simulink model "blok_net_dIt"  (R2024b)
settings: Solver=VariableStepAuto  StartTime=0.0  StopTime=10.0  RelTol=1e-3
libraries: neural x20
(part 1 of 2)
settings Model: Creator=Andrzej  LastModifiedBy=Andrzej

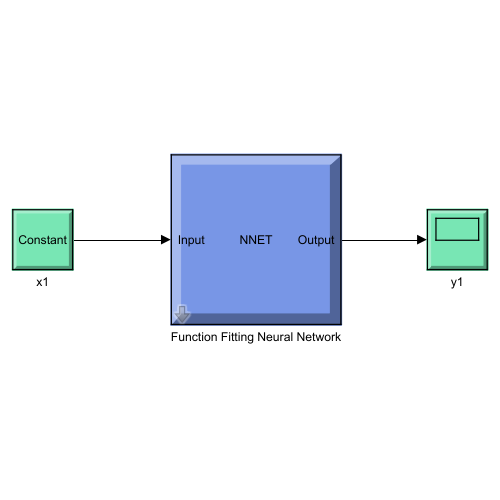
[thumbnail: Simulink's stored preview of the top-level diagram]
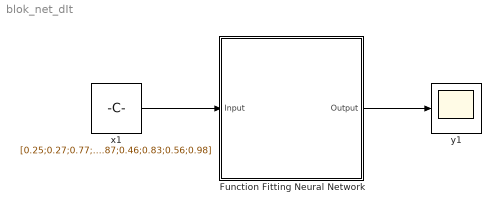
== system blok_net_dIt ==
  Function Fitting Neural Network : Subsystem
      mask help: Function Fitting Neural Network
      mask Display: e = 0.06;c1 = [120 150 230]/255;c2 = ([120 150 230]+0)/383;c3 = ([120 150 230]+128)/383;patch([0 1 1 0],[0 0 1 1],c1);patch([0 1 1 1-e 1-e 0+e],[0 0 1 1-e 0+e 0+e],c2);patch([0 0 1 1-e 0+e 0+e],[0 1 1 1-e 1-e 0+e],c3);plot([0 1 1 0 0],[0 0 1 1 0]);fprintf('NNET');port_label('input',1,' Input');port_label('output',1,'Output ');
  x1 : Constant  Value=[0.25;0.27;0.77;0.61;0.043;0.53;0.33;0.77;0.61;0.34;0.17;0.074;0.72;0.62;0.3;0.86;0.084;0.86;0.19;0.7;0.28;0.12;0.31;0.76;0.68;0.73;0.28;0.82;0.078;0.18;0.93;0.54;0.75;0.61;0.24;0.3;0.71;0.47;0.74;0.87;0.46;0.83;0.56;0.98]  SampleTime=0.1
      mask Display: e = 0.06;c1 = [120 230 180]/255;c2 = ([120 230 180]+0)/(256+128);c3 = ([120 230 180]+128)/(256+128);patch([0 1 1 0],[0 0 1 1],c1);patch([0 1 1 1-e 1-e 0+e],[0 0 1 1-e 0+e 0+e],c2);patch([0 0 1 1-e 0+e 0+e],[0 1 1 1-e 1-e 0+e],c3);plot([0 1 1 0 0],[0 0 1 1 0]);disp('Constant');
  y1 : Scope
      mask Display: e = 0.06;c1 = [120 230 180]/255;c2 = ([120 230 180]+0)/(256+128);c3 = ([120 230 180]+128)/(256+128);patch([0 1 1 0],[0 0 1 1],c1);patch([0 1 1 1-e 1-e 0+e],[0 0 1 1-e 0+e 0+e],c2);patch([0 0 1 1-e 0+e 0+e],[0 1 1 1-e 1-e 0+e],c3);plot([0 1 1 0 0],[0 0 1 1 0]);plot([0.15 0.85 0.85 0.15 0.15],[0.5 0.5 0.85 0.85 0.5]);
  wires:
  x1/1 -> Function Fitting Neural Network/1(Input)
  Function Fitting Neural Network/1(Output) -> y1/1

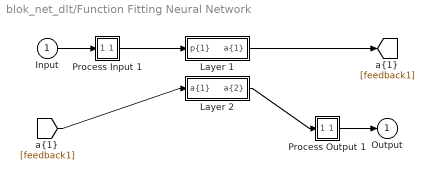
== system blok_net_dIt/Function Fitting Neural Network ==
  Input : Inport  PortDimensions=44  SampleTime=0.1
      mask Display: e = 0.06;c1 = [120 230 180]/255;c2 = ([120 230 180]+0)/(256+128);c3 = ([120 230 180]+128)/(256+128);patch([0 1 1 0],[0 0 1 1],c1);patch([0 1 1 1-e 1-e 0+e],[0 0 1 1-e 0+e 0+e],c2);patch([0 0 1 1-e 0+e 0+e],[0 1 1 1-e 1-e 0+e],c3);plot([0 1 1 0 0],[0 0 1 1 0]);
  Layer 1 : Subsystem
      mask Display: e = 0.06;c1 = [120 150 230]/255;c2 = ([120 150 230]+0)/383;c3 = ([120 150 230]+128)/383;patch([0 1 1 0],[0 0 1 1],c1);patch([0 1 1 1-e 1-e 0+e],[0 0 1 1-e 0+e 0+e],c2);patch([0 0 1 1-e 0+e 0+e],[0 1 1 1-e 1-e 0+e],c3);plot([0 1 1 0 0],[0 0 1 1 0]);
  Layer 2 : Subsystem
      mask Display: e = 0.06;c1 = [120 150 230]/255;c2 = ([120 150 230]+0)/383;c3 = ([120 150 230]+128)/383;patch([0 1 1 0],[0 0 1 1],c1);patch([0 1 1 1-e 1-e 0+e],[0 0 1 1-e 0+e 0+e],c2);patch([0 0 1 1-e 0+e 0+e],[0 1 1 1-e 1-e 0+e],c3);plot([0 1 1 0 0],[0 0 1 1 0]);
  Process Input 1 : Subsystem
      mask Display: e = 0.06;c1 = [120 150 230]/255;c2 = ([120 150 230]+0)/383;c3 = ([120 150 230]+128)/383;patch([0 1 1 0],[0 0 1 1],c1);patch([0 1 1 1-e 1-e 0+e],[0 0 1 1-e 0+e 0+e],c2);patch([0 0 1 1-e 0+e 0+e],[0 1 1 1-e 1-e 0+e],c3);plot([0 1 1 0 0],[0 0 1 1 0]);
  Process Output 1 : Subsystem
      mask Display: e = 0.06;c1 = [120 150 230]/255;c2 = ([120 150 230]+0)/383;c3 = ([120 150 230]+128)/383;patch([0 1 1 0],[0 0 1 1],c1);patch([0 1 1 1-e 1-e 0+e],[0 0 1 1-e 0+e 0+e],c2);patch([0 0 1 1-e 0+e 0+e],[0 1 1 1-e 1-e 0+e],c3);plot([0 1 1 0 0],[0 0 1 1 0]);
  Output : Outport  InitialOutput=0
      mask Display: e = 0.06;c1 = [120 230 180]/255;c2 = ([120 230 180]+0)/(256+128);c3 = ([120 230 180]+128)/(256+128);patch([0 1 1 0],[0 0 1 1],c1);patch([0 1 1 1-e 1-e 0+e],[0 0 1 1-e 0+e 0+e],c2);patch([0 0 1 1-e 0+e 0+e],[0 1 1 1-e 1-e 0+e],c3);plot([0 1 1 0 0],[0 0 1 1 0]);
  wires:
  Input/1 -> Process Input 1/1(x)
  Process Output 1/1(y) -> Output/1
  Process Input 1/1(p) -> Layer 1/1("p{1}")
  Layer 1/1("a{1}") -> [feedback1]
  [feedback1] -> Layer 2/1("a{1} ")
  Layer 2/1("a{2}") -> Process Output 1/1(a)

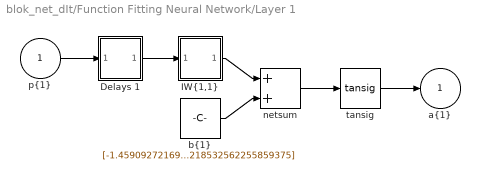
== system blok_net_dIt/Function Fitting Neural Network/Layer 1 ==
  "p{1}" : Inport  PortDimensions=44  SampleTime=0.1
      mask Display: e = 0.06;c1 = [120 230 180]/255;c2 = ([120 230 180]+0)/(256+128);c3 = ([120 230 180]+128)/(256+128);patch([0 1 1 0],[0 0 1 1],c1);patch([0 1 1 1-e 1-e 0+e],[0 0 1 1-e 0+e 0+e],c2);patch([0 0 1 1-e 0+e 0+e],[0 1 1 1-e 1-e 0+e],c3);plot([0 1 1 0 0],[0 0 1 1 0]);
  Delays 1 : Subsystem
      mask Display: e = 0.06;c1 = [120 150 230]/255;c2 = ([120 150 230]+0)/383;c3 = ([120 150 230]+128)/383;patch([0 1 1 0],[0 0 1 1],c1);patch([0 1 1 1-e 1-e 0+e],[0 0 1 1-e 0+e 0+e],c2);patch([0 0 1 1-e 0+e 0+e],[0 1 1 1-e 1-e 0+e],c3);plot([0 1 1 0 0],[0 0 1 1 0]);disp('0');
  "IW{1,1}" : Subsystem
      mask Display: e = 0.06;c1 = [120 150 230]/255;c2 = ([120 150 230]+0)/383;c3 = ([120 150 230]+128)/383;patch([0 1 1 0],[0 0 1 1],c1);patch([0 1 1 1-e 1-e 0+e],[0 0 1 1-e 0+e 0+e],c2);patch([0 0 1 1-e 0+e 0+e],[0 1 1 1-e 1-e 0+e],c3);plot([0 1 1 0 0],[0 0 1 1 0]);disp('W');
  "b{1}" : Constant  Value=[-1.4590927216917577435850716938148252665996551513671875;-1.2161094263826182082510740656289272010326385498046875;0.67240332337431407694339213776402175426483154296875;-0.57080952563055564752403370221145451068878173828125;0.5299136413583969140717044865596108138561248779296875;-0.500883856424665818707353537320159375667572021484375;0.80620597521665604556773132571834139525890350341796875;0.1146802862454827931504297566789318807423114776611328125;0.280936541276880447082220371157745830714702606201171875;0.90048946986504929679284714438836090266704559326171875;-0.26431542718953260351355538659845478832721710205078125;-0.87810750793975234085309011788922362029552459716796875;1.4374602095202082541192112330463714897632598876953125;-1.59058445523031100066191356745548546314239501953125;-1.5451182648027026456105659235618077218532562255859375]
      mask Display: e = 0.06;c1 = [120 150 230]/255;c2 = ([120 150 230]+0)/383;c3 = ([120 150 230]+128)/383;patch([0 1 1 0],[0 0 1 1],c1);patch([0 1 1 1-e 1-e 0+e],[0 0 1 1-e 0+e 0+e],c2);patch([0 0 1 1-e 0+e 0+e],[0 1 1 1-e 1-e 0+e],c3);plot([0 1 1 0 0],[0 0 1 1 0]);disp('b');
  netsum : Sum  Inputs=2  InputSameDT=on  SaturateOnIntegerOverflow=on  OutDataTypeStr=Inherit: Same as first input
      mask Display: e = 0.06;c1 = [120 150 230]/255;c2 = ([120 150 230]+0)/383;c3 = ([120 150 230]+128)/383;patch([0 1 1 0],[0 0 1 1],c1);patch([0 1 1 1-e 1-e 0+e],[0 0 1 1-e 0+e 0+e],c2);patch([0 0 1 1-e 0+e 0+e],[0 1 1 1-e 1-e 0+e],c3);plot([0 1 1 0 0],[0 0 1 1 0]);disp('+');
  tansig : neural/Transfer Functions/tansig
  "a{1}" : Outport  InitialOutput=[0;0;0;0;0;0;0;0;0;0;0;0;0;0;0]
      mask Display: e = 0.06;c1 = [120 230 180]/255;c2 = ([120 230 180]+0)/(256+128);c3 = ([120 230 180]+128)/(256+128);patch([0 1 1 0],[0 0 1 1],c1);patch([0 1 1 1-e 1-e 0+e],[0 0 1 1-e 0+e 0+e],c2);patch([0 0 1 1-e 0+e 0+e],[0 1 1 1-e 1-e 0+e],c3);plot([0 1 1 0 0],[0 0 1 1 0]);
  wires:
  "p{1}"/1 -> Delays 1/1("p{1}")
  Delays 1/1("pd{1,1}") -> "IW{1,1}"/1("pd{1,1}")
  "IW{1,1}"/1("iz{1,1}") -> netsum/1
  "b{1}"/1 -> netsum/2
  netsum/1 -> tansig/1
  tansig/1 -> "a{1}"/1

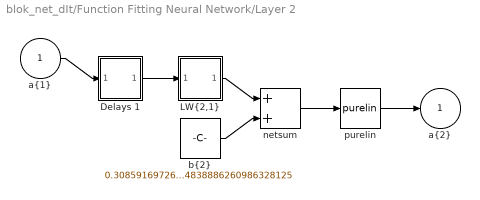
== system blok_net_dIt/Function Fitting Neural Network/Layer 2 ==
  "a{1} " : Inport  PortDimensions=15  SampleTime=0.1
      mask Display: e = 0.06;c1 = [120 230 180]/255;c2 = ([120 230 180]+0)/(256+128);c3 = ([120 230 180]+128)/(256+128);patch([0 1 1 0],[0 0 1 1],c1);patch([0 1 1 1-e 1-e 0+e],[0 0 1 1-e 0+e 0+e],c2);patch([0 0 1 1-e 0+e 0+e],[0 1 1 1-e 1-e 0+e],c3);plot([0 1 1 0 0],[0 0 1 1 0]);
  Delays 1 : Subsystem
      mask Display: e = 0.06;c1 = [120 150 230]/255;c2 = ([120 150 230]+0)/383;c3 = ([120 150 230]+128)/383;patch([0 1 1 0],[0 0 1 1],c1);patch([0 1 1 1-e 1-e 0+e],[0 0 1 1-e 0+e 0+e],c2);patch([0 0 1 1-e 0+e 0+e],[0 1 1 1-e 1-e 0+e],c3);plot([0 1 1 0 0],[0 0 1 1 0]);disp('0');
  "LW{2,1}" : Subsystem
      mask Display: e = 0.06;c1 = [120 150 230]/255;c2 = ([120 150 230]+0)/383;c3 = ([120 150 230]+128)/383;patch([0 1 1 0],[0 0 1 1],c1);patch([0 1 1 1-e 1-e 0+e],[0 0 1 1-e 0+e 0+e],c2);patch([0 0 1 1-e 0+e 0+e],[0 1 1 1-e 1-e 0+e],c3);plot([0 1 1 0 0],[0 0 1 1 0]);disp('W');
  "b{2}" : Constant  Value=0.308591697268615405835845422188867814838886260986328125
      mask Display: e = 0.06;c1 = [120 150 230]/255;c2 = ([120 150 230]+0)/383;c3 = ([120 150 230]+128)/383;patch([0 1 1 0],[0 0 1 1],c1);patch([0 1 1 1-e 1-e 0+e],[0 0 1 1-e 0+e 0+e],c2);patch([0 0 1 1-e 0+e 0+e],[0 1 1 1-e 1-e 0+e],c3);plot([0 1 1 0 0],[0 0 1 1 0]);disp('b');
  netsum : Sum  Inputs=2  InputSameDT=on  SaturateOnIntegerOverflow=on  OutDataTypeStr=Inherit: Same as first input
      mask Display: e = 0.06;c1 = [120 150 230]/255;c2 = ([120 150 230]+0)/383;c3 = ([120 150 230]+128)/383;patch([0 1 1 0],[0 0 1 1],c1);patch([0 1 1 1-e 1-e 0+e],[0 0 1 1-e 0+e 0+e],c2);patch([0 0 1 1-e 0+e 0+e],[0 1 1 1-e 1-e 0+e],c3);plot([0 1 1 0 0],[0 0 1 1 0]);disp('+');
  purelin : neural/Transfer Functions/purelin
  "a{2}" : Outport  InitialOutput=0
      mask Display: e = 0.06;c1 = [120 230 180]/255;c2 = ([120 230 180]+0)/(256+128);c3 = ([120 230 180]+128)/(256+128);patch([0 1 1 0],[0 0 1 1],c1);patch([0 1 1 1-e 1-e 0+e],[0 0 1 1-e 0+e 0+e],c2);patch([0 0 1 1-e 0+e 0+e],[0 1 1 1-e 1-e 0+e],c3);plot([0 1 1 0 0],[0 0 1 1 0]);
  wires:
  "a{1} "/1 -> Delays 1/1("p{2}")
  Delays 1/1("pd{2,1}") -> "LW{2,1}"/1("ad{2,1}")
  "LW{2,1}"/1("lz{2,1}") -> netsum/1
  "b{2}"/1 -> netsum/2
  netsum/1 -> purelin/1
  purelin/1 -> "a{2}"/1

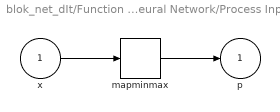
== system blok_net_dIt/Function Fitting Neural Network/Process Input 1 ==
  x : Inport  PortDimensions=44  SampleTime=0.1
      mask Display: e = 0.06;c1 = [120 230 180]/255;c2 = ([120 230 180]+0)/(256+128);c3 = ([120 230 180]+128)/(256+128);patch([0 1 1 0],[0 0 1 1],c1);patch([0 1 1 1-e 1-e 0+e],[0 0 1 1-e 0+e 0+e],c2);patch([0 0 1 1-e 0+e 0+e],[0 1 1 1-e 1-e 0+e],c3);plot([0 1 1 0 0],[0 0 1 1 0]);
  mapminmax : neural/Processing Functions/mapminmax  xmin=[200;7.5;0.0560599604440001897387446661014;0.666666670123805316094944828365;200;6.66666666666666696272613990004;0.0560599604440001897387446661014;0.666666670123805316094944828365;200;5.83333333333333303727386009996;0.0560599604440001897387446661014;0.666666670123805316094944828365;200;5;0.0560599604440001897387446661014;0.666666670123805316094944828365;200;4.16666666666666696272613990004;0.0560599604440001897387446661014;0.666666670123805316094944828365;200;3.33333333333333348136306995002;0.0560599604440001897387446661014;0.666666670123805316094944828365;200;2.5;0.0560599604440001897387446661014;0.598775219478076659029852635285;200;1.66666666666666674068153497501;0.0560599604440001897387446661014;0.444741001202892838328750713117;200;0.833333333333333370340767487505;0.0560599604440001897387446661014;0.248926720000000017973817989514;-3.66984632054533754796921130037;-3.66984632054533754796921130037;-3.66984632054533754796921130037;-3.66984632054533754796921130037;-3.66984632054533754796921130037;-3.66984632054533754796921130037;-3.66984632054533754796921130037;-3.66984632054533754796921130037]  xmax=[396.346826452357333891995949671;388.235964771228339031949872151;9.76797095137581905532897508238;1.31996715259718877533146041969;396.346826452357333891995949671;387.618095460889037440210813656;9.76797095137581905532897508238;1.31996715259718877533146041969;396.346826452357333891995949671;386.966216713948654160049045458;9.76797095137581905532897508238;1.31996715259718877533146041969;396.346826452357333891995949671;386.278944144757304002268938348;9.76797095137581905532897508238;1.31996715259718877533146041969;396.346826452357333891995949671;385.554826214493289171514334157;9.76797095137581905532897508238;1.31996715259718877533146041969;396.346826452357333891995949671;384.792340749840207081433618441;9.76797095137581905532897508238;1.31996715259718877533146041969;396.346826452357333891995949671;383.989891286615318222175119445;9.76797095137581905532897508238;1.31996715259718877533146041969;396.346826452357333891995949671;383.145803229656792154855793342;9.76797095137581905532897508238;1.31996715259718877533146041969;396.346826452357333891995949671;382.258319819841574371821479872;9.76797095137581905532897508238;1.31996715259718877533146041969;7.40930001984626951383461346268;7.40930001984626951383461346268;7.40930001984626951383461346268;7.40930001984626951383461346268;7.40930001984626951383461346268;7.40930001984626951383461346268;7.40930001984626951383461346268;7.40930001984626951383461346268]  ymin=-1  ymax=1
  p : Outport  PortDimensions=44  SampleTime=0.1
      mask Display: e = 0.06;c1 = [120 230 180]/255;c2 = ([120 230 180]+0)/(256+128);c3 = ([120 230 180]+128)/(256+128);patch([0 1 1 0],[0 0 1 1],c1);patch([0 1 1 1-e 1-e 0+e],[0 0 1 1-e 0+e 0+e],c2);patch([0 0 1 1-e 0+e 0+e],[0 1 1 1-e 1-e 0+e],c3);plot([0 1 1 0 0],[0 0 1 1 0]);
  wires:
  x/1 -> mapminmax/1
  mapminmax/1 -> p/1

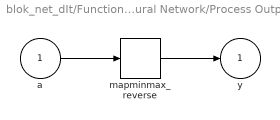
== system blok_net_dIt/Function Fitting Neural Network/Process Output 1 ==
  a : Inport  PortDimensions=1  SampleTime=0.1
      mask Display: e = 0.06;c1 = [120 230 180]/255;c2 = ([120 230 180]+0)/(256+128);c3 = ([120 230 180]+128)/(256+128);patch([0 1 1 0],[0 0 1 1],c1);patch([0 1 1 1-e 1-e 0+e],[0 0 1 1-e 0+e 0+e],c2);patch([0 0 1 1-e 0+e 0+e],[0 1 1 1-e 1-e 0+e],c3);plot([0 1 1 0 0],[0 0 1 1 0]);
  mapminmax_reverse : neural/Processing Functions/mapminmax_reverse  xmin=-0.334064474595016203117836539604  xmax=0.261856585052868462426545193011  ymin=-1  ymax=1
  y : Outport  PortDimensions=1  SampleTime=0.1
      mask Display: e = 0.06;c1 = [120 230 180]/255;c2 = ([120 230 180]+0)/(256+128);c3 = ([120 230 180]+128)/(256+128);patch([0 1 1 0],[0 0 1 1],c1);patch([0 1 1 1-e 1-e 0+e],[0 0 1 1-e 0+e 0+e],c2);patch([0 0 1 1-e 0+e 0+e],[0 1 1 1-e 1-e 0+e],c3);plot([0 1 1 0 0],[0 0 1 1 0]);
  wires:
  a/1 -> mapminmax_reverse/1
  mapminmax_reverse/1 -> y/1

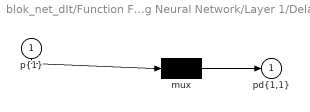
== system blok_net_dIt/Function Fitting Neural Network/Layer 1/Delays 1 ==
  "p{1}" : Inport  PortDimensions=44  SampleTime=0.1
      mask Display: e = 0.06;c1 = [120 230 180]/255;c2 = ([120 230 180]+0)/(256+128);c3 = ([120 230 180]+128)/(256+128);patch([0 1 1 0],[0 0 1 1],c1);patch([0 1 1 1-e 1-e 0+e],[0 0 1 1-e 0+e 0+e],c2);patch([0 0 1 1-e 0+e 0+e],[0 1 1 1-e 1-e 0+e],c3);plot([0 1 1 0 0],[0 0 1 1 0]);
  mux : Mux  Inputs=1
      mask Display: e = 0.06;c1 = [120 150 230]/255;c2 = ([120 150 230]+0)/383;c3 = ([120 150 230]+128)/383;patch([0 1 1 0],[0 0 1 1],c1);patch([0 1 1 1-e 1-e 0+e],[0 0 1 1-e 0+e 0+e],c2);patch([0 0 1 1-e 0+e 0+e],[0 1 1 1-e 1-e 0+e],c3);plot([0 1 1 0 0],[0 0 1 1 0]);disp('Mux')
  "pd{1,1}" : Outport
      mask Display: e = 0.06;c1 = [120 230 180]/255;c2 = ([120 230 180]+0)/(256+128);c3 = ([120 230 180]+128)/(256+128);patch([0 1 1 0],[0 0 1 1],c1);patch([0 1 1 1-e 1-e 0+e],[0 0 1 1-e 0+e 0+e],c2);patch([0 0 1 1-e 0+e 0+e],[0 1 1 1-e 1-e 0+e],c3);plot([0 1 1 0 0],[0 0 1 1 0]);
  wires:
  "p{1}"/1 -> mux/1
  mux/1 -> "pd{1,1}"/1
